simulink model "Model"  (R2025b)
settings: Solver=VariableStepAuto  StartTime=0.0  StopTime=20  RelTol=1e-3
values from neighbouring files (symbols this model uses):
  b = 0.2    [const.m]
  Cw1_x = 92    [const.m]
  Cw1_y = 96    [const.m]
  Cw1_z = 98    [const.m]
  Cw2_x = 9.2    [const.m]
  Cw2_y = 9.6    [const.m]
  Cw2_z = 9.8    [const.m]
  h1 = 0.1    [const.m]
  J_z = 126    [const.m]
  K_dv = 15    [const.m]
  L_11 = 98    [const.m]
  L_22 = 104    [const.m]
  L_66 = 125    [const.m]
  m = 110    [const.m]
  T_dv = 0.15    [const.m]
  U_max = 10    [const.m]
  V = 0.2    [const.m]
settings Model: Creator=user  LastModifiedBy=user

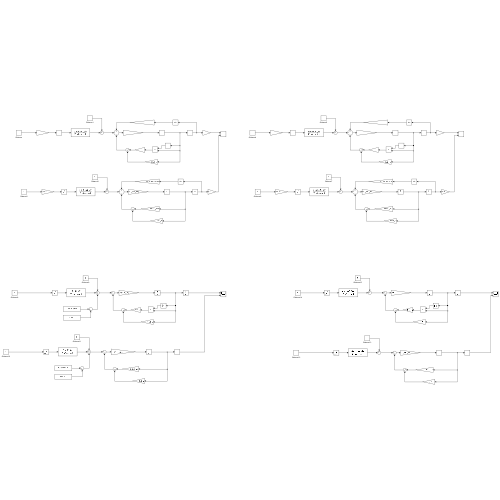
[thumbnail: Simulink's stored preview of the top-level diagram]
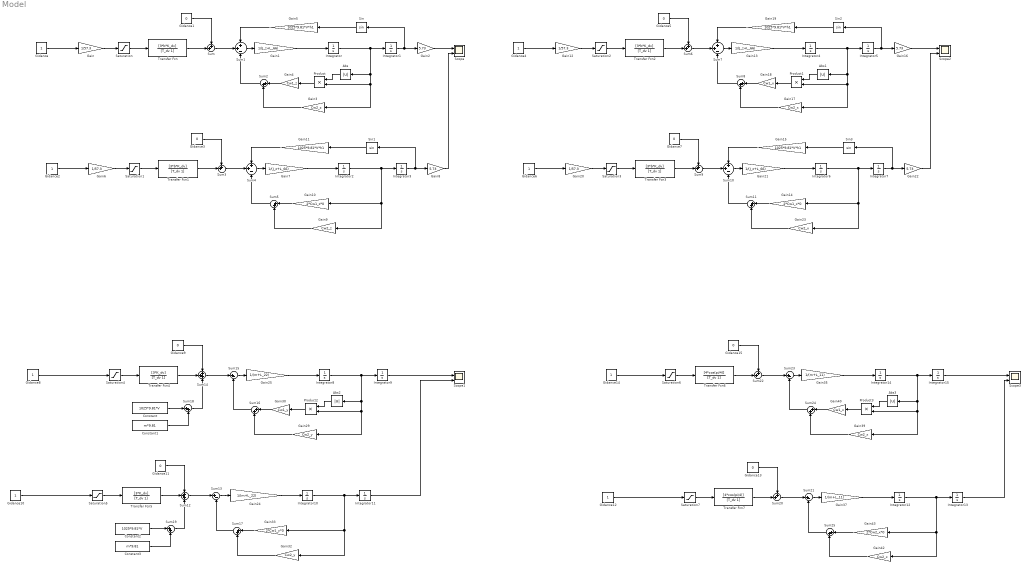
== system Model ==
  Abs{,1..3} (4 alike) : Abs  SaturateOnIntegerOverflow=off
  Constant : Constant  Value=1025*9.81*V
  Constant1 : Constant  Value=m*9.81
  Constant2 : Constant  Value=1025*9.81*V
  Constant3 : Constant  Value=m*9.81
  Gain{,6,12,20} (4 alike) : Gain  Gain=1/57.3
  Gain{1,7,13,21} (4 alike) : Gain  Gain=1/(J_z+L_66)
  Gain10 : Gain  Gain=2*Cw1_z*0
  Gain{5,11,15,19} (4 alike) : Gain  Gain=1025*9.81*V*h1
  Gain14 : Gain  Gain=2*Cw1_x*0
  Gain{2,8,16,22} (4 alike) : Gain  Gain=5.73
  Gain{17,23,39,42} (4 alike) : Gain  Gain=Cw2_x
  Gain18 : Gain  Gain=Cw1_x
  Gain24 : Gain  Gain=1/(m+L_22)
  Gain25 : Gain  Gain=1/(m+L_22)
  Gain29 : Gain  Gain=Cw2_y
  Gain3 : Gain  Gain=Cw2_z
  Gain30 : Gain  Gain=Cw1_y
  Gain32 : Gain  Gain=Cw2_y
  Gain33 : Gain  Gain=2*Cw1_y*0
  Gain35 : Gain  Gain=1/(m+L_11)
  Gain37 : Gain  Gain=1/(m+L_11)
  Gain4 : Gain  Gain=Cw1_z
  Gain40 : Gain  Gain=Cw1_x
  Gain43 : Gain  Gain=2*Cw2_x*0
  Gain9 : Gain  Gain=Cw2_z
  Gidance{,2,4,6,8,10,12,14} (8 alike) : Constant
  Gidance{1,3,5,7,9,11,13,15} (8 alike) : Constant  Value=0
  Integrator{,1..15} (16 alike) : Integrator
  Product{,1..3} (4 alike) : Product
  Saturation{,1..7} (8 alike) : Saturate  UpperLimit=U_max  LowerLimit=-U_max
  Scope{,1..3} (4 alike) : Scope  NumInputPorts=2
      Scope settings: ActiveDisplayYMinimum=-3.922067684975576  ActiveDisplayYMaximum=35.298609164780189
      Scope1 settings: ActiveDisplayYMinimum=-21017.346530471856  ActiveDisplayYMaximum=59953.208145400175
      Scope2 settings: ActiveDisplayYMinimum=-3.9403193200762421  ActiveDisplayYMaximum=35.462873880686189  DataLoggingVariableName=ScopeData2
      Scope3 settings: ActiveDisplayYMinimum=-0.10951140351601207  ActiveDisplayYMaximum=1.02640221677404  DataLoggingVariableName=ScopeData3
  Sin{,1..3} (4 alike) : Trigonometry
  Sum{,3,6,9,20,22} (6 alike) : Sum  Inputs=++|
  Sum{1,4,7,10} (4 alike) : Sum  Inputs=++-
  Sum{2,5,8,11,16..19,24..25} (10 alike) : Sum  Inputs=|++
  Sum12 : Sum  Inputs=+++
  Sum{13,15,21,23} (4 alike) : Sum  Inputs=|+-
  Sum14 : Sum  Inputs=+++
  Transfer Fcn{,1..3} (4 alike) : TransferFcn  Numerator=[3*b*K_dv]  Denominator=[T_dv 1]
  Transfer Fcn4 : TransferFcn  Numerator=[3*K_dv]  Denominator=[T_dv 1]
  Transfer Fcn5 : TransferFcn  Numerator=[3*K_dv]  Denominator=[T_dv 1]
  Transfer Fcn6 : TransferFcn  Numerator=[4*cos(pi/4)]  Denominator=[T_dv 1]
  Transfer Fcn7 : TransferFcn  Numerator=[4*cos(pi/4)]  Denominator=[T_dv 1]
  wires:
  Gidance/1 -> Gain/1
  Gain/1 -> Saturation/1
  Saturation/1 -> Transfer Fcn/1
  Transfer Fcn/1 -> Sum/2
  Gidance1/1 -> Sum/1
  Sum/1 -> Sum1/2
  Sum1/1 -> Gain1/1
  Gain1/1 -> Integrator/1
  Integrator1/1 -> Sin/1, Gain2/1
  Gain2/1 -> Scope/1
  Product/1 -> Gain4/1
  Gain4/1 -> Sum2/1
  Gain3/1 -> Sum2/2
  Abs/1 -> Product/1
  Integrator/1 -> Abs/1, Product/2, Gain3/1, Integrator1/1
  Sum2/1 -> Sum1/3
  Gain5/1 -> Sum1/1
  Sin/1 -> Gain5/1
  Sum5/1 -> Sum4/3
  Sin1/1 -> Gain11/1
  Gain7/1 -> Integrator2/1
  Sum4/1 -> Gain7/1
  Gidance3/1 -> Sum3/1
  Integrator2/1 -> Gain10/1, Gain9/1, Integrator3/1
  Gain6/1 -> Saturation1/1
  Gidance2/1 -> Gain6/1
  Gain9/1 -> Sum5/2
  Gain8/1 -> Scope/2
  Sum3/1 -> Sum4/2
  Saturation1/1 -> Transfer Fcn1/1
  Transfer Fcn1/1 -> Sum3/2
  Gain11/1 -> Sum4/1
  Gain10/1 -> Sum5/1
  Integrator3/1 -> Sin1/1, Gain8/1
  Sum8/1 -> Sum7/3
  Sin2/1 -> Gain19/1
  Abs1/1 -> Product1/1
  Gain14/1 -> Sum11/1
  Integrator7/1 -> Sin3/1, Gain22/1
  Gain15/1 -> Sum10/1
  Saturation3/1 -> Transfer Fcn3/1
  Gain22/1 -> Scope2/2
  Gain23/1 -> Sum11/2
  Sum9/1 -> Sum10/2
  Gidance6/1 -> Gain20/1
  Gain20/1 -> Saturation3/1
  Integrator6/1 -> Gain14/1, Gain23/1, Integrator7/1
  Sum10/1 -> Gain21/1
  Gidance7/1 -> Sum9/1
  Gain21/1 -> Integrator6/1
  Sin3/1 -> Gain15/1
  Gain13/1 -> Integrator4/1
  Sum7/1 -> Gain13/1
  Gidance5/1 -> Sum6/1
  Integrator4/1 -> Abs1/1, Product1/2, Gain17/1, Integrator5/1
  Gain12/1 -> Saturation2/1
  Product1/1 -> Gain18/1
  Sum11/1 -> Sum10/3
  Gidance4/1 -> Gain12/1
  Gain17/1 -> Sum8/2
  Gain16/1 -> Scope2/1
  Sum6/1 -> Sum7/2
  Saturation2/1 -> Transfer Fcn2/1
  Transfer Fcn2/1 -> Sum6/2
  Gain19/1 -> Sum7/1
  Transfer Fcn3/1 -> Sum9/2
  Gain18/1 -> Sum8/1
  Integrator5/1 -> Sin2/1, Gain16/1
  Integrator11/1 -> Scope1/2
  Transfer Fcn4/1 -> Sum14/2
  Saturation4/1 -> Transfer Fcn4/1
  Product2/1 -> Gain30/1
  Integrator9/1 -> Scope1/1
  Gain29/1 -> Sum16/2
  Sum15/1 -> Gain25/1
  Gidance9/1 -> Sum14/1
  Integrator8/1 -> Abs2/1, Product2/2, Gain29/1, Integrator9/1
  Gain25/1 -> Integrator8/1
  Gain30/1 -> Sum16/1
  Sum16/1 -> Sum15/2
  Gidance8/1 -> Saturation4/1
  Abs2/1 -> Product2/1
  Constant/1 -> Sum18/1
  Constant1/1 -> Sum18/2
  Sum18/1 -> Sum14/3
  Sum14/1 -> Sum15/1
  Constant2/1 -> Sum19/1
  Sum12/1 -> Sum13/1
  Gidance10/1 -> Saturation5/1
  Gain24/1 -> Integrator10/1
  Gain33/1 -> Sum17/1
  Gidance11/1 -> Sum12/1
  Sum17/1 -> Sum13/2
  Saturation5/1 -> Transfer Fcn5/1
  Integrator10/1 -> Gain33/1, Gain32/1, Integrator11/1
  Constant3/1 -> Sum19/2
  Transfer Fcn5/1 -> Sum12/2
  Sum19/1 -> Sum12/3
  Gain32/1 -> Sum17/2
  Sum13/1 -> Gain24/1
  Sum22/1 -> Sum23/1
  Gidance14/1 -> Saturation6/1
  Abs3/1 -> Product3/1
  Gidance15/1 -> Sum22/1
  Integrator14/1 -> Abs3/1, Product3/2, Gain39/1, Integrator15/1
  Sum24/1 -> Sum23/2
  Gain39/1 -> Sum24/2
  Saturation6/1 -> Transfer Fcn6/1
  Integrator15/1 -> Scope3/1
  Product3/1 -> Gain40/1
  Gain35/1 -> Integrator14/1
  Sum23/1 -> Gain35/1
  Transfer Fcn6/1 -> Sum22/2
  Gain40/1 -> Sum24/1
  Gidance12/1 -> Saturation7/1
  Saturation7/1 -> Transfer Fcn7/1
  Gain42/1 -> Sum25/2
  Integrator13/1 -> Scope3/2
  Integrator12/1 -> Gain43/1, Gain42/1, Integrator13/1
  Sum25/1 -> Sum21/2
  Sum20/1 -> Sum21/1
  Sum21/1 -> Gain37/1
  Transfer Fcn7/1 -> Sum20/2
  Gain37/1 -> Integrator12/1
  Gain43/1 -> Sum25/1
  Gidance13/1 -> Sum20/1
